simulink model "SwingHoldPendulumPiMod2"  (R2026b)
settings: Solver=ode1  StopTime=40  FixedStep=0.001  EnableMultiTasking=on
model workspace (MAT data in the model file):
  MQTTsample = 0.1
  PID1DD = 1.5
  PID1DI = 0.2
  PID1DP = 25
  PIDDD = 4
  PIDDI = 0.5
  PIDDP = 7
libraries: simulink x4, slpidlib x2, raspberrypiIOTlib x1
settings Model: ExtModeTrigMode=oneshot  SimulationMode=external  Creator=pawel  LastModifiedBy=super
settings SolverCC: AutoInsertRateTranBlk=on  PositivePriorityOrder=on
settings DataIOCC: ReturnWorkspaceOutputs=off  SaveFormat=Array  SignalLoggingName=sigsOut  SignalLoggingSaveFormat=ModelDataLogs
settings OptimizationCC: BlockReduction=off  BooleanDataType=off  DifferentSizesBufferReuse=on  EfficientTunableParamExpr=on  EnhancedBackFolding=on  MaxStackSize=200000  MemsetInitFltsAndDblsToZero=off  OptimizationCustomize=off  OptimizeBlockOrder=speed  PassReuseOutputArgsAs=Individual arguments  RemoveInternalMemoryZeroInit=on  RemoveRootLevelIOMemoryZeroInit=on
settings DebuggingCC: AllowSymbolicDim=off  ArithmeticOperatorsInVariantConditions=warning  FcnCallInpInsideContextMsg=warning  MergeDetectMultiDrivingBlocksExec=none  MultiTaskCondExecSysMsg=none  MultiTaskDSMMsg=warning  ParameterTunabilityLossMsg=error  SFExecutionAtInitializationDiag=none  SFNoUnconditionalDefaultTransitionDiag=warning  SFUnexpectedBacktrackingDiag=warning  SaveWithParameterizedLinksMsg=none  SignalResolutionControl=TryResolveAllWithWarning  StateNameClashWarn=warning  UnderspecifiedInitializationDetection=Classic
settings HardwareCC: ProdHWDeviceType=ARM Compatible->ARM Cortex-A (64-bit)  ProdLargestAtomicFloat=Double  ProdLargestAtomicInteger=LongLong  ProdLongLongMode=on  TargetEndianess=LittleEndian  TargetHWDeviceType=Intel->x86-64  TargetIntDivRoundTo=Zero
settings ModelReferenceCC: PropagateSignalLabelsOutOfModel=off
settings SFSimCC: CustomCodeUndefinedFunction=UseInterfaceOnly  SimUseLocalCustomCode=off
settings RTWCC: BuildConfiguration=Faster Runs  Description=Embedded Coder  HardwareBoard=Raspberry Pi (64bit)  RTWUseLocalCustomCode=off  SystemTargetFile=ert.tlc  TLCOptions="-aInlineSetEventsForThisBaseRateFcn=TLC_FALSE -aSuppressMultiTaskScheduler=TLC_FALSE  -aRateBasedStepFcn=0"  TemplateMakefile=ert_default_tmf  Toolchain=GNU GCC RPIUtils
settings CodeAppCC: ForceParamTrailComments=on  IgnoreCustomStorageClasses=off  InsertBlockDesc=on  OperatorAnnotations=on  SFDataObjDesc=on  SimulinkDataObjDesc=on
settings ERTTargetCC: CodeReplacementLibrary=ARM Cortex-A CMSIS  ExtModeIntrfLevel=Level2 - Open  ExtModeMexFile=ext_xcp  ExtModeStaticAlloc=on  SupportContinuousTime=on  SupportVariableSizeSignals=on
settings ConfigComp: CovExternalEMLEnable=off  CovSaveCumulativeToWorkspaceVar=on  CovSaveSingleToWorkspaceVar=on

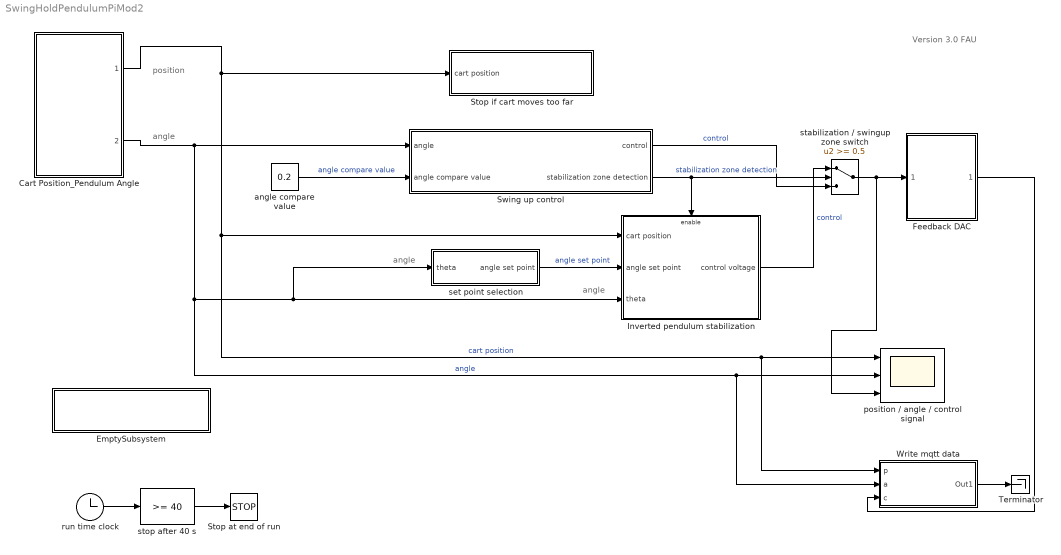
== system SwingHoldPendulumPiMod2 ==
  note: position
  note: angle
  note: Version 3.0 FAU
  note: angle
  note: angle
  Cart Position_Pendulum Angle : Subsystem  ReferencedSubsystem=CartDataReader
  EmptySubsystem : Subsystem
      mask Display:
      | image(imread('FB-inst-blue2.jpg'))
      | disp('\n\nFeedback Instruments Limited')
  Feedback DAC : Subsystem  ReferencedSubsystem=CartDataWriter  st=0.001  ch=1
  Inverted pendulum stabilization : Subsystem  TreatAsAtomicUnit=on
      mask Display:
      | image(imread('bckg.bmp'))
      | disp('Inverted pendulum \nstabilization')
  Stop at end of run : Stop
  Stop if cart moves too far : Subsystem
      mask Display:
      | image(imread('bckg.bmp'))
      | disp('Stop if cart moves too far')
  Swing up control : Subsystem
      mask Display:
      | image(imread('bckg.bmp'))
      | disp('Swing up control')
  Terminator : Terminator
  Write mqtt data : Subsystem
      mask Display: disp('MQTT Write Data\n\n PAC version 1.1')
  angle compare value : Constant  Value=0.2
  position / angle / control signal : Scope  NumInputPorts=3
      settings: SampleTime=0.001  ActiveDisplayYMinimum=-0.55  ActiveDisplayYMaximum=0.35  DataLoggingMaxPoints=100000
      mask Display: image(imread('scope.jpg'))
  run time clock : Clock
  set point selection : Subsystem
      mask Display:
      | image(imread('bckg.bmp'))
      | disp('Set point selection')
  stabilization / swingup zone switch : Switch  Threshold=0.5  SaturateOnIntegerOverflow=off  InputSameDT=off
  stop after 40 s : simulink/Logic and Bit Operations/Compare To Constant  relop=>=  const=40  OutDataTypeStr=boolean
  wires:
  Cart Position_Pendulum Angle/1 -> Inverted pendulum stabilization/1(cart position), Write mqtt data/1(p), position / angle / control signal/1, Stop if cart moves too far/1(cart position)  "cart position"
  Cart Position_Pendulum Angle/2 -> Inverted pendulum stabilization/3(theta), set point selection/1(theta), Write mqtt data/2(a), position / angle / control signal/2, Swing up control/1(angle)  "angle"
  Swing up control/1(control) -> stabilization / swingup zone switch/3  "control"
  stabilization / swingup zone switch/1 -> Feedback DAC/1, position / angle / control signal/3
  Inverted pendulum stabilization/1(control voltage) -> stabilization / swingup zone switch/1  "control"
  set point selection/1(angle set point) -> Inverted pendulum stabilization/2(angle set point)  "angle set point"
  Swing up control/2(stabilization zone detection) -> stabilization / swingup zone switch/2, Inverted pendulum stabilization/Enable  "stabilization zone detection"
  angle compare value/1 -> Swing up control/2(angle compare value)  "angle compare value"
  Write mqtt data/1(Out1) -> Terminator/1
  run time clock/1 -> stop after 40 s/1
  stop after 40 s/1 -> Stop at end of run/1
  Feedback DAC/1 -> Write mqtt data/3(c)

== system SwingHoldPendulumPiMod2/EmptySubsystem ==

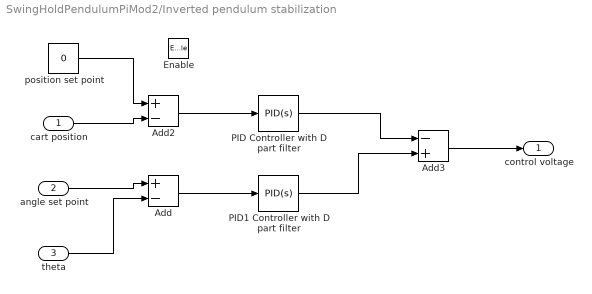
== system SwingHoldPendulumPiMod2/Inverted pendulum stabilization ==
  cart position : Inport
  angle set point : Inport  Port=2
  theta : Inport  Port=3
  Enable : EnablePort
  Add : Sum  Inputs=+-
  Add2 : Sum  Inputs=+-
  Add3 : Sum  Inputs=-+
  PID Controller with D part filter : slpidlib/PID Controller  Controller=PID  Form=Parallel  TimeDomain=Continuous-time  UseExternalTs=off  SampleTime=-1  IntegratorMethod=Forward Euler  FilterMethod=Forward Euler  ControllerParametersSource=internal  P=PIDDP  I=PIDDI  UseKiTs=off  D=PIDDD  UseExternalDerivativeSource=off  N=100  UseFilter=on  TunerSelectOption=Transfer Function Based (PID Tuner App)  InitialConditionSource=internal  InitialConditionForIntegrator=0  InitialConditionForFilter=0  DifferentiatorICPrevScaledInput=0  ExternalReset=none  TrackingMode=off  Kt=1  LimitOutput=off  SatLimitsSource=internal  UpperSaturationLimit=inf  LowerSaturationLimit=-inf  LinearizeAsGain=on  AntiWindupMode=none  Kb=1  LimitIntegrator=off  UpperIntegratorSaturationLimit=inf  LowerIntegratorSaturationLimit=-inf  POutMin=[]  POutMax=[]  IOutMin=[]  IOutMax=[]  DOutMin=[]  DOutMax=[]  NOutMin=[]  NOutMax=[]  SumOutMin=[]  SumOutMax=[]  SaturationOutMin=[]  SaturationOutMax=[]  PParamMin=[]  PParamMax=[]  IParamMin=[]  IParamMax=[]  DParamMin=[]  DParamMax=[]  NParamMin=[]  NParamMax=[]  KbParamMin=[]  KbParamMax=[]  KtParamMin=[]  KtParamMax=[]  KbOutMin=[]  KbOutMax=[]  KtOutMin=[]  KtOutMax=[]  IntegratorOutMin=[]  IntegratorOutMax=[]  FilterOutMin=[]  FilterOutMax=[]  SumI1OutMin=[]  SumI1OutMax=[]  SumI2OutMin=[]  SumI2OutMax=[]  SumI3OutMin=[]  SumI3OutMax=[]  SumI4OutMin=[]  SumI4OutMax=[]  SumDOutMin=[]  SumDOutMax=[]  DifferentiatorOutMin=[]  DifferentiatorOutMax=[]  FilterDiffOutCoefMin=[]  FilterDiffOutCoefMax=[]  ReciprocalOutMin=[]  ReciprocalOutMax=[]  SumDenOutMin=[]  SumDenOutMax=[]  SumNumOutMin=[]  SumNumOutMax=[]  DivideOutMin=[]  DivideOutMax=[]  UdiffTsProdOutMin=[]  UdiffTsProdOutMax=[]  NTsProdOutMin=[]  NTsProdOutMax=[]  UintegralTsProdOutMin=[]  UintegralTsProdOutMax=[]  UngainTsProdOutMin=[]  UngainTsProdOutMax=[]  ClampingZeroOutDataTypeStr=Inherit: Inherit via back propagation  ClampingZeroOutMin=[]  ClampingZeroOutMax=[]  FilterDenConstantOutDataTypeStr=Inherit: Inherit via back propagation  FilterDenConstantOutMin=[]  FilterDenConstantOutMax=[]  PCopyOutDataTypeStr=Inherit: Inherit via back propagation  PCopyOutMin=[]  PCopyOutMax=[]  NCopyOutDataTypeStr=Inherit: Inherit via back propagation  NCopyOutMin=[]  NCopyOutMax=[]  IntegratorContinuousStateAttributes=''  IntegratorStateMustResolveToSignalObject=off  IntegratorRTWStateStorageClass=Auto  FilterContinuousStateAttributes=''  FilterStateMustResolveToSignalObject=off  FilterRTWStateStorageClass=Auto  ParallelPVariant=InternalParameters  IdealPVariant=Disabled  IVariant=InternalParameters  DVariant=InternalParameters  IntegratorVariant=Continuous  SatVariant=Disabled  AWVariant=Passthrough  PCopyVariant=Disabled  TRVariant=Disabled  FdbkBlocksVariant=Forward  IdealPFdbkVariant=Disabled  SatFdbkVariant=Disabled  DerivativeFilterVariant=ContFilter  NVariant=InternalParameters  NCopyVariant=Disabled  FilterICVariant=InternalICsFilter  IntegratorICVariant=InternalICs  ExternalResetVariant=Disabled  TRSumVariant=Passthrough  SumFdbkVariant=Disabled  SumVariant=Sum_PID  TsampFilterVariant=InternalTs  TsampNgainVariant=Passthrough  TsampIntegralVariant=Disabled_SignalSpec  ExternalSaturationOutDataTypeStr=Inherit: Same as second input  DerivativeSourceVariant=ErrorSignal  PreIntVariant=InternalPreInt
  PID1 Controller with D part filter : slpidlib/PID Controller  Controller=PID  Form=Parallel  TimeDomain=Continuous-time  UseExternalTs=off  SampleTime=-1  IntegratorMethod=Forward Euler  FilterMethod=Forward Euler  ControllerParametersSource=internal  P=25  I=0.2  UseKiTs=off  D=1.5  UseExternalDerivativeSource=off  N=100  UseFilter=on  TunerSelectOption=Transfer Function Based (PID Tuner App)  InitialConditionSource=internal  InitialConditionForIntegrator=0  InitialConditionForFilter=0  DifferentiatorICPrevScaledInput=0  ExternalReset=none  TrackingMode=off  Kt=1  LimitOutput=off  SatLimitsSource=internal  UpperSaturationLimit=inf  LowerSaturationLimit=-inf  LinearizeAsGain=on  AntiWindupMode=none  Kb=1  LimitIntegrator=off  UpperIntegratorSaturationLimit=inf  LowerIntegratorSaturationLimit=-inf  POutMin=[]  POutMax=[]  IOutMin=[]  IOutMax=[]  DOutMin=[]  DOutMax=[]  NOutMin=[]  NOutMax=[]  SumOutMin=[]  SumOutMax=[]  SaturationOutMin=[]  SaturationOutMax=[]  PParamMin=[]  PParamMax=[]  IParamMin=[]  IParamMax=[]  DParamMin=[]  DParamMax=[]  NParamMin=[]  NParamMax=[]  KbParamMin=[]  KbParamMax=[]  KtParamMin=[]  KtParamMax=[]  KbOutMin=[]  KbOutMax=[]  KtOutMin=[]  KtOutMax=[]  IntegratorOutMin=[]  IntegratorOutMax=[]  FilterOutMin=[]  FilterOutMax=[]  SumI1OutMin=[]  SumI1OutMax=[]  SumI2OutMin=[]  SumI2OutMax=[]  SumI3OutMin=[]  SumI3OutMax=[]  SumI4OutMin=[]  SumI4OutMax=[]  SumDOutMin=[]  SumDOutMax=[]  DifferentiatorOutMin=[]  DifferentiatorOutMax=[]  FilterDiffOutCoefMin=[]  FilterDiffOutCoefMax=[]  ReciprocalOutMin=[]  ReciprocalOutMax=[]  SumDenOutMin=[]  SumDenOutMax=[]  SumNumOutMin=[]  SumNumOutMax=[]  DivideOutMin=[]  DivideOutMax=[]  UdiffTsProdOutMin=[]  UdiffTsProdOutMax=[]  NTsProdOutMin=[]  NTsProdOutMax=[]  UintegralTsProdOutMin=[]  UintegralTsProdOutMax=[]  UngainTsProdOutMin=[]  UngainTsProdOutMax=[]  ClampingZeroOutDataTypeStr=Inherit: Inherit via back propagation  ClampingZeroOutMin=[]  ClampingZeroOutMax=[]  FilterDenConstantOutDataTypeStr=Inherit: Inherit via back propagation  FilterDenConstantOutMin=[]  FilterDenConstantOutMax=[]  PCopyOutDataTypeStr=Inherit: Inherit via back propagation  PCopyOutMin=[]  PCopyOutMax=[]  NCopyOutDataTypeStr=Inherit: Inherit via back propagation  NCopyOutMin=[]  NCopyOutMax=[]  IntegratorContinuousStateAttributes=''  IntegratorStateMustResolveToSignalObject=off  IntegratorRTWStateStorageClass=Auto  FilterContinuousStateAttributes=''  FilterStateMustResolveToSignalObject=off  FilterRTWStateStorageClass=Auto  ParallelPVariant=InternalParameters  IdealPVariant=Disabled  IVariant=InternalParameters  DVariant=InternalParameters  IntegratorVariant=Continuous  SatVariant=Disabled  AWVariant=Passthrough  PCopyVariant=Disabled  TRVariant=Disabled  FdbkBlocksVariant=Forward  IdealPFdbkVariant=Disabled  SatFdbkVariant=Disabled  DerivativeFilterVariant=ContFilter  NVariant=InternalParameters  NCopyVariant=Disabled  FilterICVariant=InternalICsFilter  IntegratorICVariant=InternalICs  ExternalResetVariant=Disabled  TRSumVariant=Passthrough  SumFdbkVariant=Disabled  SumVariant=Sum_PID  TsampFilterVariant=InternalTs  TsampNgainVariant=Passthrough  TsampIntegralVariant=Disabled_SignalSpec  ExternalSaturationOutDataTypeStr=Inherit: Same as second input  DerivativeSourceVariant=ErrorSignal  PreIntVariant=InternalPreInt
  position set point : Constant  Value=0
  control voltage : Outport
  wires:
  PID1 Controller with D part filter/1 -> Add3/2
  Add/1 -> PID1 Controller with D part filter/1
  position set point/1 -> Add2/1
  Add2/1 -> PID Controller with D part filter/1
  PID Controller with D part filter/1 -> Add3/1
  cart position/1 -> Add2/2
  theta/1 -> Add/2
  angle set point/1 -> Add/1
  Add3/1 -> control voltage/1

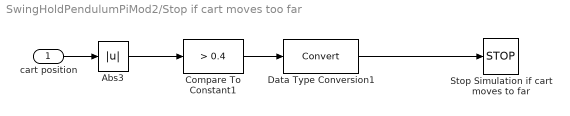
== system SwingHoldPendulumPiMod2/Stop if cart moves too far ==
  cart position : Inport
  Abs3 : Abs  SaturateOnIntegerOverflow=off
  Compare To Constant1 : simulink/Logic and Bit Operations/Compare To Constant  relop=>  const=0.4  OutDataTypeStr=boolean  ZeroCross=off
  Data Type Conversion1 : DataTypeConversion  SaturateOnIntegerOverflow=off  RndMeth=Floor
  Stop Simulation if cart moves to far : Stop
  wires:
  cart position/1 -> Abs3/1
  Data Type Conversion1/1 -> Stop Simulation if cart moves to far/1
  Compare To Constant1/1 -> Data Type Conversion1/1
  Abs3/1 -> Compare To Constant1/1

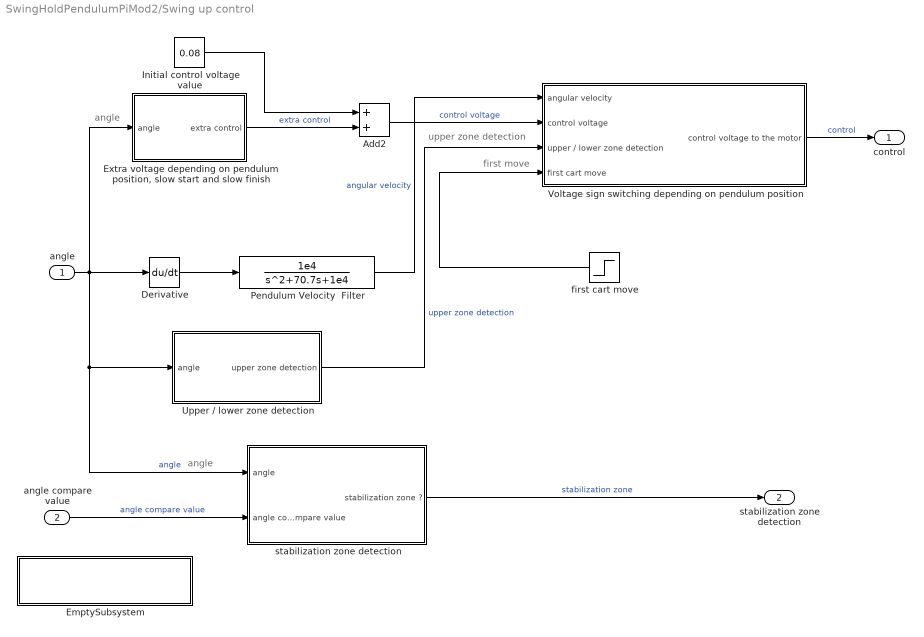
== system SwingHoldPendulumPiMod2/Swing up control ==
  note: angle
  note: angle
  note: upper zone detection
  note: first move
  angle : Inport
  angle compare value : Inport  Port=2
  Add2 : Sum
  Derivative : Derivative
  EmptySubsystem : Subsystem
      mask Display:
      | image(imread('FB-inst-blue2.jpg'))
      | disp('\n\nFeedback Instruments Limited')
  "Extra voltage depending on pendulum position, slow start and slow finish" : Subsystem
      mask Display:
      | image(imread('bckg.bmp'))
      | disp('Extra voltage')
  Initial control voltage value : Constant  Value=0.08
  Pendulum Velocity  Filter : TransferFcn  Numerator=[1e4]  Denominator=[1 70.7 1e4]
  Upper / lower zone detection : Subsystem
      mask Display:
      | image(imread('bckg.bmp'))
      | disp('Upper / lower zone \ndetection')
  Voltage sign switching depending on pendulum position : Subsystem
      mask Display:
      | image(imread('bckg.bmp'))
      | disp('Voltage sign switching \ndepending on pendulum position')
  first cart move : Step  Time=0.3  InitialValue=-0.3  FinalValue=0  SampleTime=0
  "stabilization zone detection " : Subsystem
      mask Display:
      | image(imread('bckg.bmp'))
      | disp('stabilization zone detection')
  control : Outport
  stabilization zone detection : Outport  Port=2
  wires:
  Upper / lower zone detection/1(upper zone detection) -> Voltage sign switching depending on pendulum position/3(upper / lower zone detection)  "upper zone detection"
  Initial control voltage value/1 -> Add2/1
  "Extra voltage depending on pendulum position, slow start and slow finish"/1(extra control) -> Add2/2  "extra control"
  Voltage sign switching depending on pendulum position/1(control voltage to the motor) -> control/1  "control"
  first cart move/1 -> Voltage sign switching depending on pendulum position/4(first cart move)
  Add2/1 -> Voltage sign switching depending on pendulum position/2(control voltage)  "control voltage"
  angle/1 -> "Extra voltage depending on pendulum position, slow start and slow finish"/1(angle), Derivative/1, "stabilization zone detection "/1(angle), Upper / lower zone detection/1(angle)  "angle"
  Pendulum Velocity  Filter/1 -> Voltage sign switching depending on pendulum position/1(angular velocity)  "angular velocity"
  "stabilization zone detection "/1(stabilization zone ?) -> stabilization zone detection/1  "stabilization zone"
  angle compare value/1 -> "stabilization zone detection "/2(angle compare value)  "angle compare value"
  Derivative/1 -> Pendulum Velocity  Filter/1

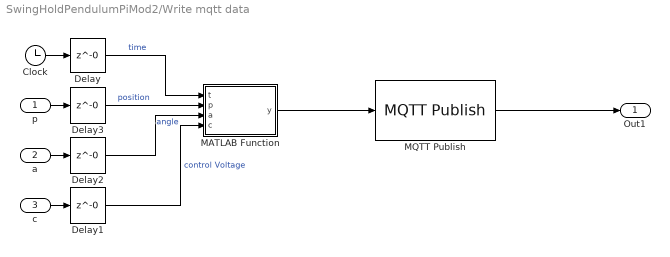
== system SwingHoldPendulumPiMod2/Write mqtt data ==
  p : Inport
  a : Inport  Port=2
  c : Inport  Port=3
  Clock : Clock
  Delay{,1..3} (4 alike) : Delay  DelayLength=0  InitialCondition=0  SampleTime=MQTTsample
  MATLAB Function : MATLAB Function  TreatAsAtomicUnit=on
  MQTT Publish : raspberrypiIOTlib/MQTT Publish  Topic=raspi/to_django  QoS=0  RetainMsg=off  blockPlatform=RASPBERRYPI
  Out1 : Outport
  wires:
  MQTT Publish/1 -> Out1/1
  a/1 -> Delay2/1
  Clock/1 -> Delay/1
  Delay/1 -> MATLAB Function/1(t)  "time"
  p/1 -> Delay3/1
  Delay2/1 -> MATLAB Function/3(a)  "angle"
  c/1 -> Delay1/1
  Delay1/1 -> MATLAB Function/4(c)  "control Voltage"
  MATLAB Function/1(y) -> MQTT Publish/1
  Delay3/1 -> MATLAB Function/2(p)  "position"

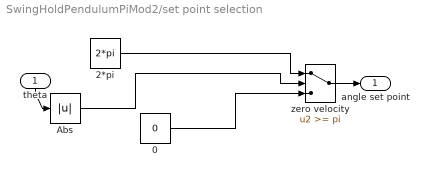
== system SwingHoldPendulumPiMod2/set point selection ==
  theta : Inport
  0 : Constant  Value=0
  2*pi : Constant  Value=2*pi
  Abs : Abs  SaturateOnIntegerOverflow=off
  zero velocity : Switch  Threshold=pi  SaturateOnIntegerOverflow=off  InputSameDT=off
  angle set point : Outport
  wires:
  zero velocity/1 -> angle set point/1
  theta/1 -> Abs/1
  Abs/1 -> zero velocity/2
  2*pi/1 -> zero velocity/1
  0/1 -> zero velocity/3

== system SwingHoldPendulumPiMod2/Swing up control/EmptySubsystem ==

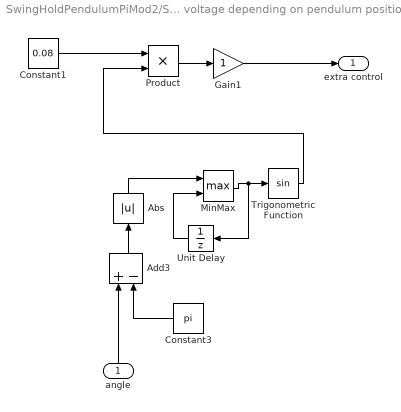
== system SwingHoldPendulumPiMod2/Swing up control/Extra voltage depending on pendulum position, slow start and slow finish ==
  angle : Inport
  Abs : Abs  SaturateOnIntegerOverflow=off
  Add3 : Sum  Inputs=+-
  Constant1 : Constant  Value=0.08
  Constant3 : Constant  Value=pi
  Gain1 : Gain
  MinMax : MinMax  Function=max  Inputs=2
  Product : Product  RndMeth=Zero
  Trigonometric Function : Trigonometry
  Unit Delay : UnitDelay  SampleTime=0.01
  extra control : Outport
  wires:
  Product/1 -> Gain1/1
  Constant1/1 -> Product/1
  Constant3/1 -> Add3/2
  Add3/1 -> Abs/1
  Abs/1 -> MinMax/1
  MinMax/1 -> Trigonometric Function/1, Unit Delay/1
  Unit Delay/1 -> MinMax/2
  angle/1 -> Add3/1
  Gain1/1 -> extra control/1
  Trigonometric Function/1 -> Product/2

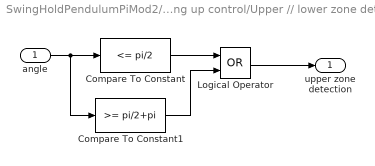
== system SwingHoldPendulumPiMod2/Swing up control/Upper // lower zone detection ==
  angle : Inport
  Compare To Constant : simulink/Logic and Bit Operations/Compare To Constant  relop=<=  const=pi/2  OutDataTypeStr=uint8  ZeroCross=off
  Compare To Constant1 : simulink/Logic and Bit Operations/Compare To Constant  relop=>=  const=pi/2+pi  OutDataTypeStr=uint8  ZeroCross=off
  Logical Operator : Logic  Operator=OR  AllPortsSameDT=off  OutDataTypeStr=boolean
  upper zone detection : Outport
  wires:
  Logical Operator/1 -> upper zone detection/1
  angle/1 -> Compare To Constant1/1, Compare To Constant/1
  Compare To Constant1/1 -> Logical Operator/2
  Compare To Constant/1 -> Logical Operator/1

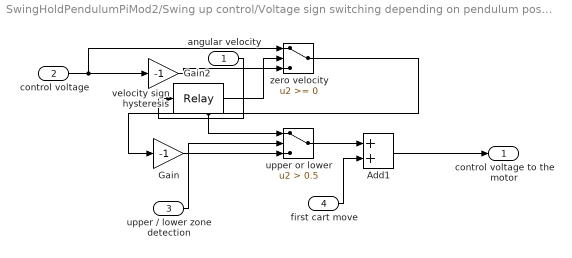
== system SwingHoldPendulumPiMod2/Swing up control/Voltage sign switching depending on pendulum position ==
  angular velocity : Inport
  control voltage : Inport  Port=2
  upper / lower zone detection : Inport  Port=3
  first cart move : Inport  Port=4
  Add1 : Sum
  Gain : Gain  Gain=-1
  Gain2 : Gain  Gain=-1
  upper or lower : Switch  Criteria=u2 > Threshold  Threshold=0.5  SaturateOnIntegerOverflow=off  InputSameDT=off
  velocity sign hysteresis : Relay  OnSwitchValue=0.3  OffSwitchValue=-0.3  OffOutputValue=-1
  zero velocity : Switch  SaturateOnIntegerOverflow=off  InputSameDT=off
  control voltage to the motor : Outport
  wires:
  Gain/1 -> upper or lower/3
  zero velocity/1 -> upper or lower/1, Gain/1
  control voltage/1 -> zero velocity/1, Gain2/1
  Gain2/1 -> zero velocity/3
  upper or lower/1 -> Add1/1
  upper / lower zone detection/1 -> upper or lower/2
  Add1/1 -> control voltage to the motor/1
  first cart move/1 -> Add1/2
  angular velocity/1 -> velocity sign hysteresis/1
  velocity sign hysteresis/1 -> zero velocity/2

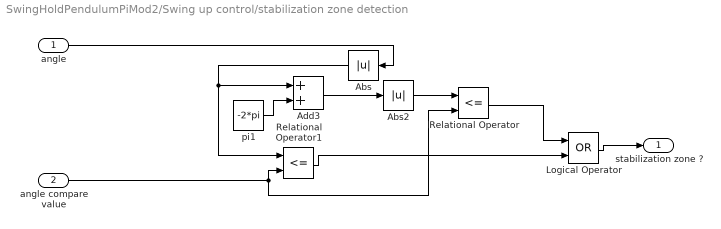
== system SwingHoldPendulumPiMod2/Swing up control/stabilization zone detection  ==
  angle : Inport
  angle compare value : Inport  Port=2
  Abs : Abs  SaturateOnIntegerOverflow=off
  Abs2 : Abs  SaturateOnIntegerOverflow=off
  Add3 : Sum
  Logical Operator : Logic  Operator=OR  AllPortsSameDT=off  OutDataTypeStr=boolean
  Relational Operator : RelationalOperator  Operator=<=  OutDataTypeStr=boolean  InputSameDT=off
  Relational Operator1 : RelationalOperator  Operator=<=  OutDataTypeStr=boolean  InputSameDT=off
  pi1 : Constant  Value=-2*pi
  stabilization zone ? : Outport
  wires:
  angle compare value/1 -> Relational Operator/2, Relational Operator1/2
  Logical Operator/1 -> stabilization zone ?/1
  angle/1 -> Abs/1
  Abs2/1 -> Relational Operator/1
  Relational Operator/1 -> Logical Operator/1
  Add3/1 -> Abs2/1
  pi1/1 -> Add3/2
  Relational Operator1/1 -> Logical Operator/2
  Abs/1 -> Relational Operator1/1, Add3/1

== matlab function SwingHoldPendulumPiMod2/Write mqtt data/MATLAB Function ==
  data: t input; p input; y output; a input; c input
function y = fmtstr(t,p,a,c)
% One sprintf: the append/num2str version compiled to an empty MQTT payload.
% angle wrapped to (-pi, pi]: 0 = upright, +-pi = hanging. c is the command sent to the ESP32.
a = -(mod(-a + pi, 2*pi) - pi);
y = string(sprintf('{"time": "%.3f", "position": "%.4f", "angle": "%.4f", "control": "%.3f"}', t, p, a, c));
end
